simulink model "Body3DOF_VDB"  (R2023a)
settings: Solver=VariableStepAuto  StartTime=0.0  StopTime=10  MaxStep=0.002  RelTol=1e-6
undefined symbols (not defined in the file): l_f, l_r, m
libraries: autolibshared x1
settings Model: Creator=Tan_Tram  LastModifiedBy=Tan_Tram

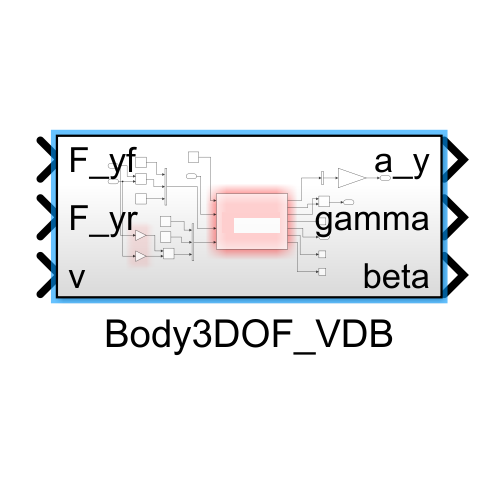
[thumbnail: Simulink's stored preview of the top-level diagram]
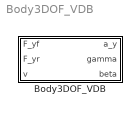
== system Body3DOF_VDB ==
  Body3DOF_VDB : Subsystem

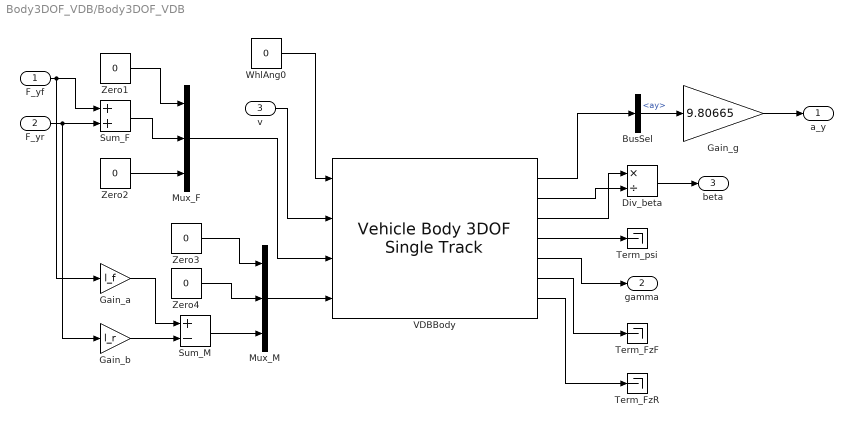
== system Body3DOF_VDB/Body3DOF_VDB ==
  F_yf : Inport
  F_yr : Inport  Port=2
  v : Inport  Port=3
  BusSel : BusSelector  OutputSignals=BdyFrm.Cg.Acc.ay
  Div_beta : Product  Inputs=*/
  Gain_a : Gain  Gain=l_f
  Gain_b : Gain  Gain=l_r
  Gain_g : Gain  Gain=9.80665
  Mux_F : Mux  Inputs=3
  Mux_M : Mux  Inputs=3
  Sum_F : Sum
  Sum_M : Sum  Inputs=+-
  Term_FzF : Terminator
  Term_FzR : Terminator
  Term_psi : Terminator
  VDBBody : autolibshared/Vehicle Body 3DOF Single Track  trackMode=Single (bicycle)  inputMode=External longitudinal velocity  frontSteerMode=on  rearSteerMode=off  windMode=off  muMode=off  extFMode=on  extMMode=on  htchFMode=off  htchMMode=off  extXo=off  extpsio=off  extxdoto=off  extro=off  extYo=off  extTamb=off  extydoto=off  aMode=2  NF=2  NR=2  m=m  a=l_f  b=l_r  h=0.35  dh=1  hh=0.2  X_o=0  xdot_o=vdb_v0  CalphaMode=off  sigmaMode=off  d=0  hl=0  w=[1.4,1.4]  Cy_f=0  Cy_r=0  sigma_f=.1  sigma_r=.1  alpha_f_brk=[-.1 .1]  Cy_f_data=[-9e3 9e3]  alpha_r_brk=[-.1 .1]  Cy_r_data=[-9e3 9e3]  Y_o=0  ydot_o=0  Izz=Iz  psi_o=0  r_o=0  Af=2  Cd=0  Cl=0  Cpm=0  beta_w=[0 0.01:0.01:0.3]  Cs=[0 0 0 0 0 0 0 0 0 0 0 0 0 0 0 0 0 0 0 0 0 0 0 0 0 0 0 0 0 0 0]  Cym=[0 0 0 0 0 0 0 0 0 0 0 0 0 0 0 0 0 0 0 0 0 0 0 0 0 0 0 0 0 0 0]  Pabs=101325  Tair=273  g=9.81  mu=1  xdot_tol=.01  Fznom=5000  Fxtire_sat=7e4  Fytire_sat=7e4  longOff=0  latOff=0  vertOff=0  wrapAng=off
  WhlAng0 : Constant  Value=0
  Zero{1..4} (4 alike) : Constant  Value=0
  a_y : Outport
  gamma : Outport  Port=2
  beta : Outport  Port=3
  wires:
  Zero4/1 -> Mux_M/2
  Zero3/1 -> Mux_M/1
  Zero1/1 -> Mux_F/1
  Zero2/1 -> Mux_F/3
  v/1 -> VDBBody/2
  F_yf/1 -> Gain_a/1, Sum_F/1
  F_yr/1 -> Sum_F/2, Gain_b/1
  Sum_M/1 -> Mux_M/3
  Sum_F/1 -> Mux_F/2
  Gain_a/1 -> Sum_M/1
  Gain_b/1 -> Sum_M/2
  Mux_F/1 -> VDBBody/3
  WhlAng0/1 -> VDBBody/1
  Mux_M/1 -> VDBBody/4
  VDBBody/1 -> BusSel/1
  VDBBody/2 -> Div_beta/2
  VDBBody/3 -> Div_beta/1
  VDBBody/5 -> gamma/1
  VDBBody/4 -> Term_psi/1
  VDBBody/7 -> Term_FzR/1
  VDBBody/6 -> Term_FzF/1
  Div_beta/1 -> beta/1
  BusSel/1 -> Gain_g/1  "<ay>"
  Gain_g/1 -> a_y/1
